simulink model "Simulaciones_de_Control"  (R2026b)
settings: Solver=ode15s  StopTime=3  MaxStep=1e-3
values from neighbouring files (symbols this model uses):
  alpha_Cu = 3.9e-3    (= 0.0039)    [coeficientes.m]
  b_eq = b_m + b_l/(r^2)    (= 2.19444444444e-05)    [coeficientes.m]
  C_ts = 0.818    [coeficientes.m]
  g = 9.80665    [coeficientes.m]
  init_I0 = 0    [coeficientes.m]
  init_Id = 0    [coeficientes.m]
  init_Iq = 0    [coeficientes.m]
  init_theta = 0    [coeficientes.m]
  init_Ts = 20    [coeficientes.m]
  init_w = 0    [coeficientes.m]
  J_eq = J_m + J_l/(r^2)    (= 4.58263888889e-05)    [coeficientes.m]
  K_et = 2*p_obs    (= 6400)    [coeficientes.m]
  K_ew = p_obs^2    (= 10240000)    [coeficientes.m]
  k_l = k_l_min + m_l*l_l    (= 1)    [coeficientes.m]
  Kd_mov = wn_mov * (2*zeta_mov + 1) * J_eq    (= 0.0916527777778)    [coeficientes.m]
  Ki_mov = wn_mov^3 * J_eq    (= 23463.1111111)    [coeficientes.m]
  Kp_mov = wn_mov^2 * (2*zeta_mov + 1) * J_eq    (= 73.3222222222)    [coeficientes.m]
  L_d = 6.6e-3    (= 0.0066)    [coeficientes.m]
  L_ls = 0.8e-3    (= 0.0008)    [coeficientes.m]
  L_q = 5.8e-3    (= 0.0058)    [coeficientes.m]
  lambda = 0.016    [coeficientes.m]
  Pp = 3    [coeficientes.m]
  r = 120.0    (= 120)    [coeficientes.m]
  R_sREF = 1.02    [coeficientes.m]
  R_tsamb = 146.7    [coeficientes.m]
  T_amb = 20    [coeficientes.m]
  T_sREF = 20    [coeficientes.m]
libraries: eeTransforms x12
(part 2 of 2)

== system Simulaciones_de_Control/Subsystem Reference1/Transformada Inversa de Park ==
  θm : Inport
  Vd : Inport  Port=2
  Vq : Inport  Port=3
  V0 : Inport  Port=4
  Bus Creator : BusCreator  Inputs=3
  Bus Creator1 : BusCreator  Inputs=3
  Demux : Demux  Outputs=3
  Gain3 : Gain  Gain=Pp
  Inverse Park Transform : eeTransforms/Inverse Park Transform  AxisAlignment=Q-axis  PowerInvariant=off
      settings: LibrarySourceBlock=|
      | ee_sl_lib/Mathematical
      | Transforms/Inverse
      | Park Transform
  Vdq0 : Outport
  Vabc : Outport  Port=2
  wires:
  Gain3/1 -> Inverse Park Transform/2
  Inverse Park Transform/1 -> Demux/1  "v_abc"
  Demux/1 -> Bus Creator/1  "Va"
  Demux/3 -> Bus Creator/3  "Vc"
  Demux/2 -> Bus Creator/2  "Vb"
  Bus Creator/1 -> Vabc/1
  θm/1 -> Gain3/1
  Vd/1 -> Bus Creator1/1
  Vq/1 -> Bus Creator1/2
  V0/1 -> Bus Creator1/3
  Bus Creator1/1 -> Vdq0/1, Inverse Park Transform/1

== system Simulaciones_de_Control/Subsystem Reference1/Transformada_Directa_de_Park_I ==
  Iabc : Inport  OutDataTypeStr=Bus: Iabc
  θm : Inport  Port=2
  Bus Creator : BusCreator  Inputs=3
  Demux : Demux  Outputs=3
  Gain3 : Gain  Gain=Pp
  Park Transform : eeTransforms/Park Transform  AxisAlignment=Q-axis  PowerInvariant=off
      settings: LibrarySourceBlock=|
      | ee_sl_lib/Mathematical
      | Transforms/Park Transform
  Idq0 : Outport  OutDataTypeStr=Bus: Idq0
  wires:
  Gain3/1 -> Park Transform/2
  Park Transform/1 -> Demux/1  "Idq0"
  Demux/1 -> Bus Creator/1  "Id"
  Demux/3 -> Bus Creator/3  "I0"
  Demux/2 -> Bus Creator/2  "Iq"
  Bus Creator/1 -> Idq0/1
  Iabc/1 -> Park Transform/1
  θm/1 -> Gain3/1

== system Simulaciones_de_Control/Subsystem Reference2/Estimador de Estado Reducido ==
  T*m : Inport
  θm : Inport  Port=2
  Gain : Gain  Gain=1/J_eq
  Gain1 : Gain  Gain=K_ew
  Gain2 : Gain  Gain=K_et
  Integrator : Integrator
  Integrator1 : Integrator
  Sum : Sum  Inputs=|++
  Sum1 : Sum  Inputs=|++
  Sum2 : Sum  Inputs=+-
  ~ωm : Outport
  ~θm : Outport  Port=2
  wires:
  T*m/1 -> Gain/1
  Gain/1 -> Sum/1
  Sum/1 -> Integrator/1  "~dωm"
  Sum1/1 -> Integrator1/1  "~ωm+e*K_et"
  Integrator/1 -> ~ωm/1, Sum1/1  "~ωm"
  Gain1/1 -> Sum/2
  Gain2/1 -> Sum1/2
  Sum2/1 -> Gain1/1, Gain2/1  "eθ"
  θm/1 -> Sum2/1  "θm"
  Integrator1/1 -> ~θm/1, Sum2/2  "~θm"

== system Simulaciones_de_Control/Subsystem Reference2/Modulador de Torque Equivalente ==
  T°s : Inport
  ωm : Inport  Port=2
  Iabc : Inport  Port=3
  θm : Inport  Port=4
  T*m : Inport  Port=5
  dinamicRs? : Inport  Port=6
  T°ref : Inport  Port=7
  Constant1 : Constant  Value=g
  Constant2 : Constant  Value=T_sREF
  Constant3 : Constant
  Gain : Gain  Gain=alpha_Cu
  Gain1 : Gain  Gain=R_sREF
  Ground : Ground
  Lazo de Control de Corrientes Virtuales : Subsystem  ReferencedSubsystem=Lazo_Corrientes
      settings: PortSchema="{\"entries\":[{\"content\":{\"sides\":[{\"content\":{\"connectorIds\":[\"In2\",\"In3\",\"In1\",\"In4\",\"In5\"]},\"type\":\"ConnectorPlacement.EquallySpacedRectSide\",\"uuid\":\"7378df2b-1b9c-42cd-9ef6-9bfa4de31228\"},{\"content\":{\"connectorIds\":[\"Out2\",\"Out1\",\"Out3\"],\"side\":\"RIGHT\"},\"type\":\"ConnectorPlacement.EquallySpacedRectSide\",\"uuid\":\"75ac4e09-b611-4ee2-aa1e-16791f3f98b8\"},{\"content\":{\"side\":\"TOP\"},\"type\":\"ConnectorPlacement.EquallySpacedRectSide\",\"uuid\":\"c32b7829-5b6a-417b-8aae-eaa4caf59bef\"}]},\"type\":\"ConnectorPlacement.EquallySpacedConnector\",\"uuid\":\"1d84f5ff-db01-492a-bfe1-22065b3eebb0\"}],\"packageUris\":[\"http://schema.mathworks.com/mf0/Connector/R2020b\"],\"version\":\"1.0\"}"
  Modulador de Tensiones Virtuales : Subsystem  ReferencedSubsystem=Modulador_Tensiones
      settings: PortSchema="{\"entries\":[{\"content\":{\"sides\":[{\"content\":{\"connectorIds\":[\"In2\",\"In1\",\"In3\",\"In6\",\"In7\",\"In5\",\"In4\"]},\"type\":\"ConnectorPlacement.EquallySpacedRectSide\",\"uuid\":\"561a625a-719f-47d4-85d3-a88e423068dd\"},{\"content\":{\"connectorIds\":[\"Out2\",\"Out1\"],\"side\":\"RIGHT\"},\"type\":\"ConnectorPlacement.EquallySpacedRectSide\",\"uuid\":\"c1cdd74a-6c1d-470e-a6ac-8d72e83b5cc5\"},{\"content\":{\"side\":\"TOP\"},\"type\":\"ConnectorPlacement.EquallySpacedRectSide\",\"uuid\":\"c5935c6f-534c-46b9-aa64-6d6dabbbb210\"}]},\"type\":\"ConnectorPlacement.EquallySpacedConnector\",\"uuid\":\"b0debde9-6e18-4e06-b0c4-28c9c51e472d\"}],\"packageUris\":[\"http://schema.mathworks.com/mf0/Connector/R2020b\"],\"version\":\"1.0\"}"
  Modulador y Compensación de Torque : Subsystem  ReferencedSubsystem=Lazo_Torque
      settings: PortSchema="{\"entries\":[{\"content\":{\"sides\":[{\"content\":{\"connectorIds\":[\"In5\",\"In1\",\"In2\",\"In3\",\"In4\"]},\"type\":\"ConnectorPlacement.EquallySpacedRectSide\",\"uuid\":\"ea9ad4ab-f607-4d37-9442-85f6cfda2486\"},{\"content\":{\"connectorIds\":[\"Out1\"],\"side\":\"RIGHT\"},\"type\":\"ConnectorPlacement.EquallySpacedRectSide\",\"uuid\":\"696b5fe5-1f6c-4fc9-932e-86b56d49996f\"},{\"content\":{\"side\":\"TOP\"},\"type\":\"ConnectorPlacement.EquallySpacedRectSide\",\"uuid\":\"45e3ac4c-5a2f-4a79-9454-e497b07295c7\"}]},\"type\":\"ConnectorPlacement.EquallySpacedConnector\",\"uuid\":\"ad401c21-3c60-4ab4-96eb-f449fc93609a\"}],\"packageUris\":[\"http://schema.mathworks.com/mf0/Connector/R2020b\"],\"version\":\"1.0\"}"
  Subsystem : Subsystem
  Sum : Sum  Inputs=|+-
  Sum1 : Sum  Inputs=|++
  Switch : Switch  Criteria=u2 > Threshold  SaturateOnIntegerOverflow=off  InputSameDT=off
  Vabc : Outport
  Vdq0 : Outport  Port=2
  wires:
  Sum1/1 -> Gain1/1
  Constant3/1 -> Sum1/2
  Gain/1 -> Sum1/1
  Sum/1 -> Gain/1
  Constant2/1 -> Sum/2
  T°ref/1 -> Sum/1
  Constant1/1 -> Modulador y Compensación de Torque/5
  Modulador de Tensiones Virtuales/2 -> Vdq0/1
  Gain1/1 -> Switch/3
  Switch/1 -> Modulador de Tensiones Virtuales/4  "Rs"
  dinamicRs?/1 -> Switch/2  "True_False"
  Subsystem/1(R_s) -> Switch/1  "Rs"
  T°s/1 -> Subsystem/1(T°s)
  Iabc/1 -> Modulador y Compensación de Torque/2, Lazo de Control de Corrientes Virtuales/4, Modulador de Tensiones Virtuales/6  "Iabc"
  Ground/1 -> Lazo de Control de Corrientes Virtuales/3, Lazo de Control de Corrientes Virtuales/2
  Modulador de Tensiones Virtuales/1 -> Vabc/1
  ωm/1 -> Modulador y Compensación de Torque/4, Modulador de Tensiones Virtuales/5  "ωm"
  θm/1 -> Modulador y Compensación de Torque/3, Lazo de Control de Corrientes Virtuales/5, Modulador de Tensiones Virtuales/7  "θm"
  T*m/1 -> Modulador y Compensación de Torque/1
  Modulador y Compensación de Torque/1 -> Lazo de Control de Corrientes Virtuales/1
  Lazo de Control de Corrientes Virtuales/3 -> Modulador de Tensiones Virtuales/3
  Lazo de Control de Corrientes Virtuales/2 -> Modulador de Tensiones Virtuales/2
  Lazo de Control de Corrientes Virtuales/1 -> Modulador de Tensiones Virtuales/1

== system Simulaciones_de_Control/Subsystem Reference2/PID Movimiento ==
  ωm : Inport  Unit=rad/s
  θm : Inport  Port=2
  θm* : Inport  Port=3  Unit=rad/s
  ωm* : Inport  Port=4  Unit=rad/s
  Gain : Gain  Gain=Kd_mov
  Gain1 : Gain  Gain=Kp_mov
  Gain2 : Gain  Gain=Ki_mov
  Integrator1 : Integrator
  Sum : Sum  Inputs=|+-
  Sum1 : Sum  Inputs=+++
  Sum2 : Sum  Inputs=|+-
  T*m : Outport
  wires:
  Gain1/1 -> Sum1/2
  Sum1/1 -> T*m/1
  Gain2/1 -> Sum1/1
  Gain/1 -> Sum1/3
  θm*/1 -> Sum2/1
  Sum/1 -> Gain/1  "eω"
  θm/1 -> Sum2/2
  ωm*/1 -> Sum/1
  ωm/1 -> Sum/2
  Integrator1/1 -> Gain2/1  "e∫θ"
  Sum2/1 -> Gain1/1, Integrator1/1  "eθ"

== system Simulaciones_de_Control/Subsystem Reference2/Planta (Modelo Global No Lineal) ==
  note: Sistema Global No Lineal
  Vabc : Inport  OutDataTypeStr=Bus: Vabc
  T_ld : Inport  Port=2
  g : Inport  Port=3
  T°amb : Inport  Port=4
  Id(0) : Inport  Port=5
  Bus Selector : BusSelector  OutputSignals=Vd,Vq,V0
  Gain : Gain  Gain=Pp
  Subsistema Electromagnetico : Subsystem
  Subsistema Mecanico Equivalente : Subsystem
  Subsistema Termico : Subsystem
  Transformada Directa de Park : Subsystem
  Transformada Inversa de Park : Subsystem  ReferencedSubsystem=Transformada_Inversa_de_Park_I
  θm : Outport
  Iabc : Outport  Port=2  OutDataTypeStr=Bus: Iabc
  T°s : Outport  Port=3
  ωm : Outport  Port=4
  Tm : Outport  Port=5
  wires:
  Id(0)/1 -> Subsistema Electromagnetico/6(Id(0))
  Transformada Inversa de Park/1 -> Iabc/1  "Iabc"
  Bus Selector/3 -> Subsistema Electromagnetico/5(V0)  "<V0>"
  Bus Selector/2 -> Subsistema Electromagnetico/4(Vq)  "<Vq>"
  Bus Selector/1 -> Subsistema Electromagnetico/3(Vd)  "<Vd>"
  Transformada Directa de Park/1(Vdq0) -> Bus Selector/1
  g/1 -> Subsistema Mecanico Equivalente/3(g)
  T°amb/1 -> Subsistema Termico/2(T°amb)
  Vabc/1 -> Transformada Directa de Park/1(Vabc)
  T_ld/1 -> Subsistema Mecanico Equivalente/2(T_ld)
  Gain/1 -> Subsistema Electromagnetico/2(ωr)
  Subsistema Termico/1(R_s) -> Subsistema Electromagnetico/1(R_s)
  Subsistema Electromagnetico/2(T_m) -> Tm/1, Subsistema Mecanico Equivalente/1(T_m)  "Tm"
  Subsistema Mecanico Equivalente/2(θm) -> θm/1, Transformada Inversa de Park/2, Transformada Directa de Park/2(θm)  "θm"
  Subsistema Mecanico Equivalente/1(ωm) -> ωm/1, Gain/1  "ωm"
  Subsistema Electromagnetico/1(Idq0) -> Transformada Inversa de Park/1, Subsistema Termico/1(Idq0)  "Idq0"
  Subsistema Termico/2(T°s) -> T°s/1  "T°s"

== system Simulaciones_de_Control/Subsystem Reference2/Sensores Ideales ==
  note: RTD
  note: Amperimetros
  note: Encoder
  θm : Inport
  Iabc : Inport  Port=2
  T°s : Inport  Port=3
  Bus Creator : BusCreator  Inputs=3
  Bus Selector : BusSelector  OutputSignals=Ia,Ib,Ic
  Gain{,1..4} (5 alike) : Gain
  θm' : Outport
  Iabc' : Outport  Port=2
  T°s' : Outport  Port=3
  wires:
  Gain3/1 -> Bus Creator/3  "Ic"
  Gain1/1 -> Bus Creator/1  "Ia"
  Gain2/1 -> Bus Creator/2  "Ib"
  Bus Selector/3 -> Gain3/1  "<Ic>"
  Bus Selector/2 -> Gain2/1  "<Ib>"
  Bus Selector/1 -> Gain1/1  "<Ia>"
  Iabc/1 -> Bus Selector/1
  Bus Creator/1 -> Iabc'/1
  Gain4/1 -> T°s'/1
  T°s/1 -> Gain4/1
  Gain/1 -> θm'/1
  θm/1 -> Gain/1

== system Simulaciones_de_Control/Subsystem Reference2/Transformada_Directa_de_Park_I ==
  Iabc : Inport  OutDataTypeStr=Bus: Iabc
  θm : Inport  Port=2
  Ancho_abc : SignalSpecification  Dimensions=3
  Bus Creator : BusCreator  Inputs=3
  Bus to Vector : BusToVector
  Demux : Demux  Outputs=3
  Gain3 : Gain  Gain=Pp
  Park Transform : eeTransforms/Park Transform  AxisAlignment=Q-axis  PowerInvariant=off
      settings: LibrarySourceBlock=|
      | ee_sl_lib/Mathematical
      | Transforms/Park Transform
  Idq0 : Outport  OutDataTypeStr=Bus: Idq0
  wires:
  Ancho_abc/1 -> Park Transform/1
  Bus to Vector/1 -> Ancho_abc/1
  θm/1 -> Gain3/1
  Iabc/1 -> Bus to Vector/1
  Bus Creator/1 -> Idq0/1
  Demux/2 -> Bus Creator/2  "Iq"
  Demux/3 -> Bus Creator/3  "I0"
  Demux/1 -> Bus Creator/1  "Id"
  Park Transform/1 -> Demux/1  "Idq0"
  Gain3/1 -> Park Transform/2

== system Simulaciones_de_Control/Simulacion Modulador de Tension/Modulador de Tensiones Virtuales/Transformada Directa de Park ==
  Iabc : Inport
  θm : Inport  Port=2
  Bus Creator : BusCreator  Inputs=3
  Demux : Demux  Outputs=3
  Gain3 : Gain  Gain=Pp
  Park Transform : eeTransforms/Park Transform  AxisAlignment=Q-axis  PowerInvariant=off
      settings: LibrarySourceBlock=|
      | ee_sl_lib/Mathematical
      | Transforms/Park Transform
  Idq0 : Outport
  wires:
  Gain3/1 -> Park Transform/2
  Park Transform/1 -> Demux/1  "Idq0"
  Demux/1 -> Bus Creator/1  "Id"
  Demux/3 -> Bus Creator/3  "I0"
  Demux/2 -> Bus Creator/2  "Iq"
  Bus Creator/1 -> Idq0/1
  Iabc/1 -> Park Transform/1
  θm/1 -> Gain3/1

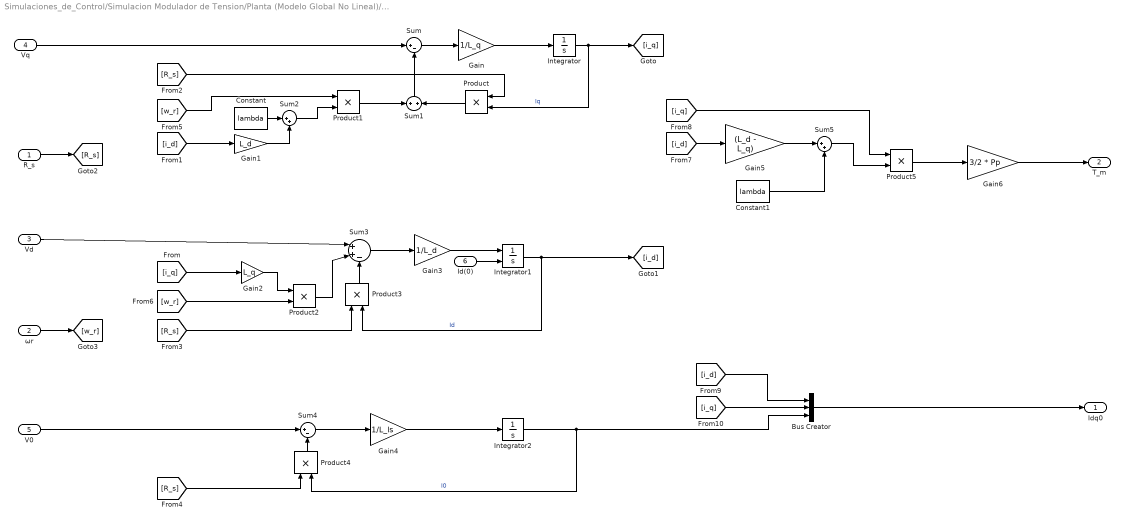
== system Simulaciones_de_Control/Simulacion Modulador de Tension/Planta (Modelo Global No Lineal)/Subsistema Electromagnetico ==
  R_s : Inport
  ωr : Inport  Port=2
  Vd : Inport  Port=3
  Vq : Inport  Port=4
  V0 : Inport  Port=5
  Id(0) : Inport  Port=6
  Bus Creator : BusCreator  Inputs=3
  Constant : Constant  Value=lambda
  Constant1 : Constant  Value=lambda
  Gain : Gain  Gain=1/L_q
  Gain1 : Gain  Gain=L_d
  Gain2 : Gain  Gain=L_q
  Gain3 : Gain  Gain=1/L_d
  Gain4 : Gain  Gain=1/L_ls
  Gain5 : Gain  Gain=(L_d - L_q)
  Gain6 : Gain  Gain=3/2 * Pp
  Integrator : Integrator  InitialCondition=init_Iq
  Integrator1 : Integrator  InitialConditionSource=external  InitialCondition=init_Id
  Integrator2 : Integrator  InitialCondition=init_I0
  Product{,1..5} (6 alike) : Product
  Sum : Sum  Inputs=|+-
  Sum1 : Sum
  Sum2 : Sum  Inputs=|++
  Sum3 : Sum  Inputs=|++-
  Sum4 : Sum  Inputs=|+-
  Sum5 : Sum  Inputs=|++
  Idq0 : Outport
  T_m : Outport  Port=2
  wires:
  [i_q] -> Bus Creator/2
  [i_d] -> Bus Creator/1
  Id(0)/1 -> Integrator1/2
  Bus Creator/1 -> Idq0/1
  [i_q] -> Product5/1
  [i_d] -> Gain5/1
  [w_r] -> Product1/1
  ωr/1 -> [w_r]
  [R_s] -> Product4/1
  [R_s] -> Product3/1
  R_s/1 -> [R_s]
  [i_d] -> Gain1/1
  Gain6/1 -> T_m/1
  Product5/1 -> Gain6/1
  Constant1/1 -> Sum5/2
  Integrator1/1 -> Product3/2, [i_d]  "Id"
  Sum5/1 -> Product5/2
  Gain5/1 -> Sum5/1
  V0/1 -> Sum4/1
  Sum4/1 -> Gain4/1
  Gain4/1 -> Integrator2/1
  Integrator2/1 -> Product4/2, Bus Creator/3  "I0"
  Product4/1 -> Sum4/2
  Vd/1 -> Sum3/1
  Sum3/1 -> Gain3/1
  Gain3/1 -> Integrator1/1
  Product3/1 -> Sum3/3
  Gain/1 -> Integrator/1
  Vq/1 -> Sum/1
  Sum/1 -> Gain/1
  Constant/1 -> Sum2/1
  Sum2/1 -> Product1/2
  Gain1/1 -> Sum2/2
  Product1/1 -> Sum1/1
  Sum1/1 -> Sum/2
  Product/1 -> Sum1/2
  [R_s] -> Product/1
  Integrator/1 -> [i_q], Product/2  "Iq"
  [i_q] -> Gain2/1
  Product2/1 -> Sum3/2
  Gain2/1 -> Product2/1
  [w_r] -> Product2/2

== system Simulaciones_de_Control/Simulacion Modulador de Tension/Planta (Modelo Global No Lineal)/Subsistema Mecanico Equivalente ==
  note: $\theta_m$
  note: $\omega_m$
  note: $\dot{\omega}_m$
  note: $T_{ld}$
  note: $T_m$
  T_m : Inport
  T_ld : Inport  Port=2
  g : Inport  Port=3
  Gain : Gain  Gain=1/r
  Gain1 : Gain  Gain=b_eq
  Gain2 : Gain  Gain=k_l/r
  Gain3 : Gain  Gain=1/J_eq
  Gain4 : Gain  Gain=1/r
  Integrator : Integrator  InitialCondition=init_w
  Integrator1 : Integrator  InitialCondition=init_theta
  Product : Product
  Sin : Trigonometry
  Sum : Sum  Inputs=|+-
  Sum1 : Sum  Inputs=+++
  ωm : Outport
  θm : Outport  Port=2
  wires:
  Integrator1/1 -> θm/1, Gain4/1
  Integrator/1 -> Gain1/1, Integrator1/1, ωm/1
  g/1 -> Product/1
  Product/1 -> Sum1/2
  T_ld/1 -> Gain/1
  Gain4/1 -> Sin/1
  Gain3/1 -> Integrator/1
  Gain1/1 -> Sum1/3
  Sin/1 -> Gain2/1
  Gain/1 -> Sum1/1
  Gain2/1 -> Product/2
  Sum1/1 -> Sum/2
  T_m/1 -> Sum/1
  Sum/1 -> Gain3/1

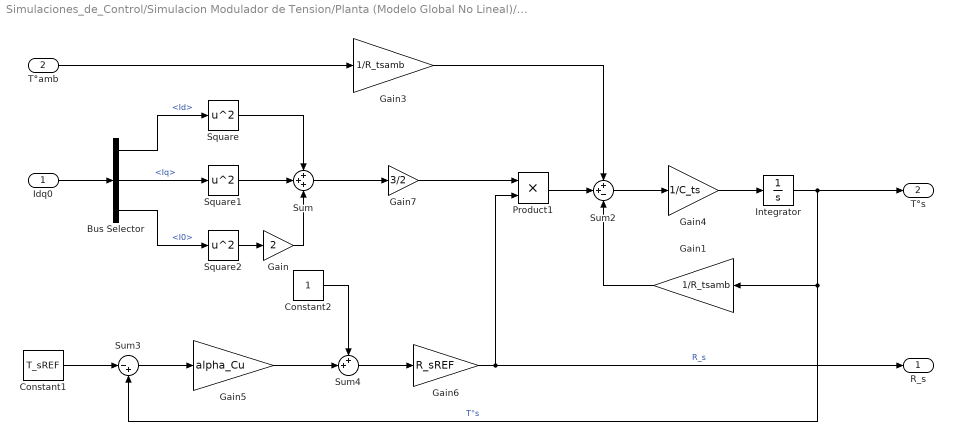
== system Simulaciones_de_Control/Simulacion Modulador de Tension/Planta (Modelo Global No Lineal)/Subsistema Termico ==
  Idq0 : Inport
  T°amb : Inport  Port=2
  Bus Selector : BusSelector  OutputSignals=Id,Iq,I0
  Constant1 : Constant  Value=T_sREF
  Constant2 : Constant
  Gain : Gain  Gain=2
  Gain1 : Gain  Gain=1/R_tsamb
  Gain3 : Gain  Gain=1/R_tsamb
  Gain4 : Gain  Gain=1/C_ts
  Gain5 : Gain  Gain=alpha_Cu
  Gain6 : Gain  Gain=R_sREF
  Gain7 : Gain  Gain=3/2
  Integrator : Integrator  InitialCondition=init_Ts
  Product1 : Product
  Square : Math  Operator=square
  Square1 : Math  Operator=square
  Square2 : Math  Operator=square
  Sum : Sum  Inputs=+++
  Sum2 : Sum  Inputs=++-
  Sum3 : Sum  Inputs=|-+
  Sum4 : Sum  Inputs=++|
  R_s : Outport
  T°s : Outport  Port=2
  wires:
  Bus Selector/3 -> Square2/1  "<I0>"
  Bus Selector/1 -> Square/1  "<Id>"
  Constant2/1 -> Sum4/1
  Idq0/1 -> Bus Selector/1
  Gain3/1 -> Sum2/1
  Gain1/1 -> Sum2/3
  Gain4/1 -> Integrator/1
  Product1/1 -> Sum2/2
  Square/1 -> Sum/1
  Sum2/1 -> Gain4/1
  Square2/1 -> Gain/1
  Sum/1 -> Gain7/1
  T°amb/1 -> Gain3/1
  Sum3/1 -> Gain5/1
  Gain5/1 -> Sum4/2
  Gain/1 -> Sum/3
  Constant1/1 -> Sum3/1
  Sum4/1 -> Gain6/1
  Gain7/1 -> Product1/1
  Gain6/1 -> Product1/2, R_s/1  "R_s"
  Integrator/1 -> T°s/1, Gain1/1, Sum3/2  "T°s"
  Square1/1 -> Sum/2
  Bus Selector/2 -> Square1/1  "<Iq>"

== system Simulaciones_de_Control/Subsystem Reference/Modulador de Torque Equivalente/Subsystem ==
  T°s : Inport
  Constant1 : Constant  Value=T_sREF
  Constant2 : Constant
  Gain5 : Gain  Gain=alpha_Cu
  Gain6 : Gain  Gain=R_sREF
  Sum3 : Sum  Inputs=+-|
  Sum4 : Sum  Inputs=|++
  R_s : Outport
  wires:
  T°s/1 -> Sum3/1
  Gain5/1 -> Sum4/1
  Gain6/1 -> R_s/1  "R_s"
  Constant1/1 -> Sum3/2
  Constant2/1 -> Sum4/2
  Sum4/1 -> Gain6/1
  Sum3/1 -> Gain5/1

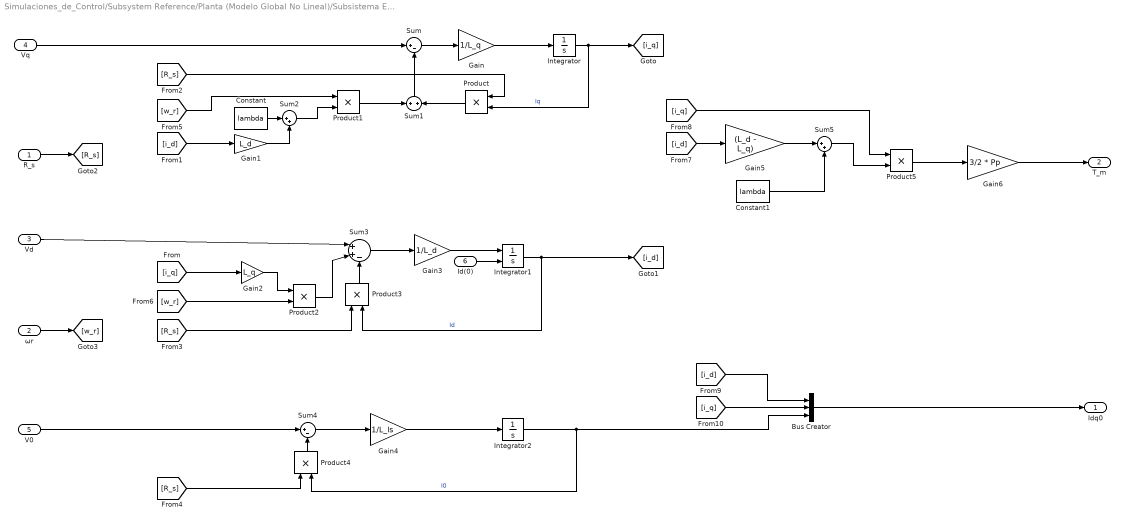
== system Simulaciones_de_Control/Subsystem Reference/Planta (Modelo Global No Lineal)/Subsistema Electromagnetico ==
  R_s : Inport
  ωr : Inport  Port=2
  Vd : Inport  Port=3
  Vq : Inport  Port=4
  V0 : Inport  Port=5
  Id(0) : Inport  Port=6
  Bus Creator : BusCreator  Inputs=3
  Constant : Constant  Value=lambda
  Constant1 : Constant  Value=lambda
  Gain : Gain  Gain=1/L_q
  Gain1 : Gain  Gain=L_d
  Gain2 : Gain  Gain=L_q
  Gain3 : Gain  Gain=1/L_d
  Gain4 : Gain  Gain=1/L_ls
  Gain5 : Gain  Gain=(L_d - L_q)
  Gain6 : Gain  Gain=3/2 * Pp
  Integrator : Integrator  InitialCondition=init_Iq
  Integrator1 : Integrator  InitialConditionSource=external  InitialCondition=init_Id
  Integrator2 : Integrator  InitialCondition=init_I0
  Product{,1..5} (6 alike) : Product
  Sum : Sum  Inputs=|+-
  Sum1 : Sum
  Sum2 : Sum  Inputs=|++
  Sum3 : Sum  Inputs=|++-
  Sum4 : Sum  Inputs=|+-
  Sum5 : Sum  Inputs=|++
  Idq0 : Outport
  T_m : Outport  Port=2
  wires:
  [w_r] -> Product2/2
  Gain2/1 -> Product2/1
  Product2/1 -> Sum3/2
  [i_q] -> Gain2/1
  Integrator/1 -> Product/2, [i_q]  "Iq"
  [R_s] -> Product/1
  Product/1 -> Sum1/2
  Sum1/1 -> Sum/2
  Product1/1 -> Sum1/1
  Gain1/1 -> Sum2/2
  Sum2/1 -> Product1/2
  Constant/1 -> Sum2/1
  Sum/1 -> Gain/1
  Vq/1 -> Sum/1
  Gain/1 -> Integrator/1
  Product3/1 -> Sum3/3
  Gain3/1 -> Integrator1/1
  Sum3/1 -> Gain3/1
  Vd/1 -> Sum3/1
  Product4/1 -> Sum4/2
  Integrator2/1 -> Bus Creator/3, Product4/2  "I0"
  Gain4/1 -> Integrator2/1
  Sum4/1 -> Gain4/1
  V0/1 -> Sum4/1
  Gain5/1 -> Sum5/1
  Sum5/1 -> Product5/2
  Integrator1/1 -> [i_d], Product3/2  "Id"
  Constant1/1 -> Sum5/2
  Product5/1 -> Gain6/1
  Gain6/1 -> T_m/1
  [i_d] -> Gain1/1
  R_s/1 -> [R_s]
  [R_s] -> Product3/1
  [R_s] -> Product4/1
  ωr/1 -> [w_r]
  [w_r] -> Product1/1
  [i_d] -> Gain5/1
  [i_q] -> Product5/1
  Bus Creator/1 -> Idq0/1
  Id(0)/1 -> Integrator1/2
  [i_d] -> Bus Creator/1
  [i_q] -> Bus Creator/2

== system Simulaciones_de_Control/Subsystem Reference/Planta (Modelo Global No Lineal)/Subsistema Mecanico Equivalente ==
  note: $T_m$
  note: $T_{ld}$
  note: $\dot{\omega}_m$
  note: $\omega_m$
  note: $\theta_m$
  T_m : Inport
  T_ld : Inport  Port=2
  g : Inport  Port=3
  Gain : Gain  Gain=1/r
  Gain1 : Gain  Gain=b_eq
  Gain2 : Gain  Gain=k_l/r
  Gain3 : Gain  Gain=1/J_eq
  Gain4 : Gain  Gain=1/r
  Integrator : Integrator  InitialCondition=init_w
  Integrator1 : Integrator  InitialCondition=init_theta
  Product : Product
  Sin : Trigonometry
  Sum : Sum  Inputs=|+-
  Sum1 : Sum  Inputs=+++
  ωm : Outport
  θm : Outport  Port=2
  wires:
  Sum/1 -> Gain3/1
  T_m/1 -> Sum/1
  Sum1/1 -> Sum/2
  Gain2/1 -> Product/2
  Gain/1 -> Sum1/1
  Sin/1 -> Gain2/1
  Gain1/1 -> Sum1/3
  Gain3/1 -> Integrator/1
  Gain4/1 -> Sin/1
  T_ld/1 -> Gain/1
  Product/1 -> Sum1/2
  g/1 -> Product/1
  Integrator/1 -> ωm/1, Integrator1/1, Gain1/1
  Integrator1/1 -> Gain4/1, θm/1

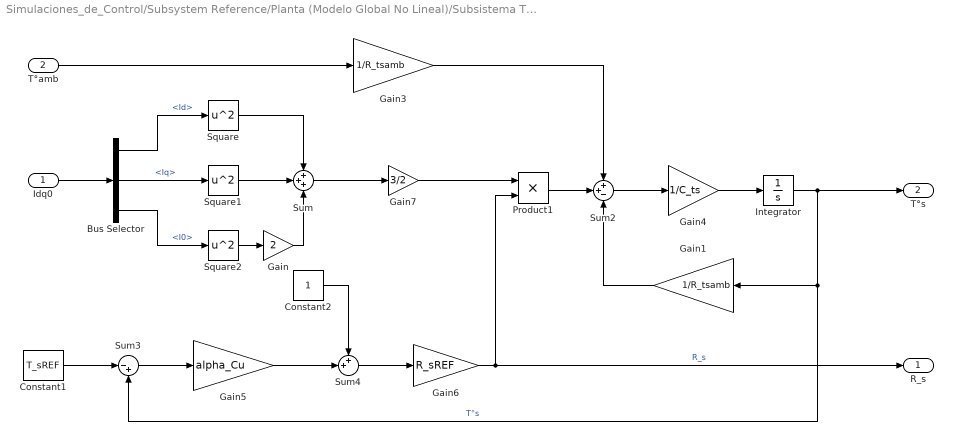
== system Simulaciones_de_Control/Subsystem Reference/Planta (Modelo Global No Lineal)/Subsistema Termico ==
  Idq0 : Inport
  T°amb : Inport  Port=2
  Bus Selector : BusSelector  OutputSignals=Id,Iq,I0
  Constant1 : Constant  Value=T_sREF
  Constant2 : Constant
  Gain : Gain  Gain=2
  Gain1 : Gain  Gain=1/R_tsamb
  Gain3 : Gain  Gain=1/R_tsamb
  Gain4 : Gain  Gain=1/C_ts
  Gain5 : Gain  Gain=alpha_Cu
  Gain6 : Gain  Gain=R_sREF
  Gain7 : Gain  Gain=3/2
  Integrator : Integrator  InitialCondition=init_Ts
  Product1 : Product
  Square : Math  Operator=square
  Square1 : Math  Operator=square
  Square2 : Math  Operator=square
  Sum : Sum  Inputs=+++
  Sum2 : Sum  Inputs=++-
  Sum3 : Sum  Inputs=|-+
  Sum4 : Sum  Inputs=++|
  R_s : Outport
  T°s : Outport  Port=2
  wires:
  Bus Selector/2 -> Square1/1  "<Iq>"
  Square1/1 -> Sum/2
  Integrator/1 -> Sum3/2, Gain1/1, T°s/1  "T°s"
  Gain6/1 -> R_s/1, Product1/2  "R_s"
  Gain7/1 -> Product1/1
  Sum4/1 -> Gain6/1
  Constant1/1 -> Sum3/1
  Gain/1 -> Sum/3
  Gain5/1 -> Sum4/2
  Sum3/1 -> Gain5/1
  T°amb/1 -> Gain3/1
  Sum/1 -> Gain7/1
  Square2/1 -> Gain/1
  Sum2/1 -> Gain4/1
  Square/1 -> Sum/1
  Product1/1 -> Sum2/2
  Gain4/1 -> Integrator/1
  Gain1/1 -> Sum2/3
  Gain3/1 -> Sum2/1
  Idq0/1 -> Bus Selector/1
  Constant2/1 -> Sum4/1
  Bus Selector/1 -> Square/1  "<Id>"
  Bus Selector/3 -> Square2/1  "<I0>"

== system Simulaciones_de_Control/Subsystem Reference/Planta (Modelo Global No Lineal)/Transformada Directa de Park ==
  Vabc : Inport  OutDataTypeStr=Bus: Vabc
  θm : Inport  Port=2
  Bus Creator : BusCreator  Inputs=3
  Demux : Demux  Outputs=3
  Gain3 : Gain  Gain=Pp
  MATLAB Function2 : MATLAB Function  Commented=on  TreatAsAtomicUnit=on
  Park Transform : eeTransforms/Park Transform  AxisAlignment=Q-axis  PowerInvariant=off
      settings: LibrarySourceBlock=|
      | ee_sl_lib/Mathematical
      | Transforms/Park Transform
  Vdq0 : Outport  OutDataTypeStr=Bus: Vdq0
  wires:
  Vabc/1 -> Park Transform/1
  Park Transform/1 -> Demux/1  "v_dq0"
  θm/1 -> Gain3/1
  Bus Creator/1 -> Vdq0/1
  Demux/2 -> Bus Creator/2  "Vq"
  Demux/3 -> Bus Creator/3  "V0"
  Demux/1 -> Bus Creator/1  "Vd"
  Gain3/1 -> Park Transform/2

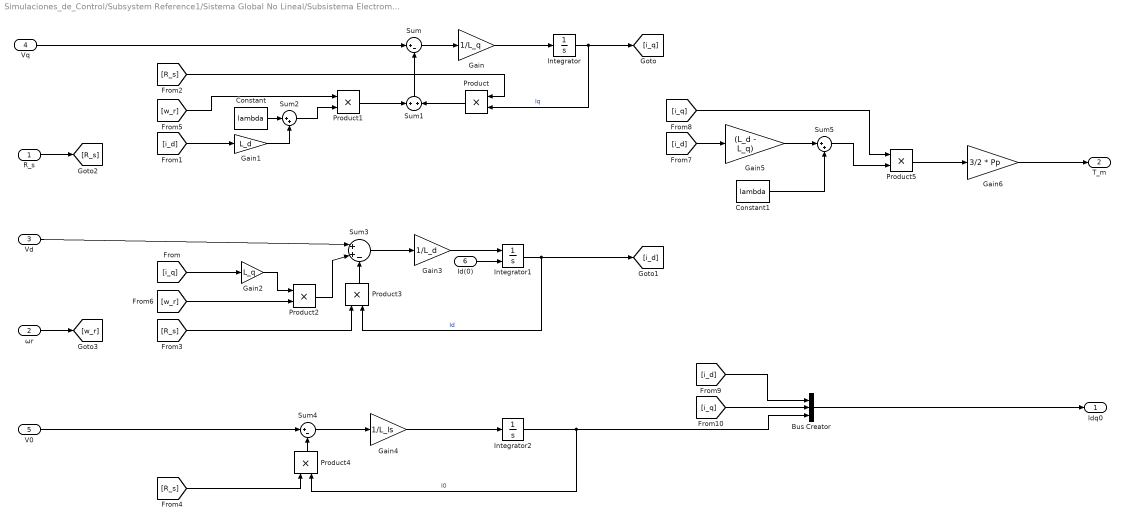
== system Simulaciones_de_Control/Subsystem Reference1/Sistema Global No Lineal/Subsistema Electromagnetico ==
  R_s : Inport
  ωr : Inport  Port=2
  Vd : Inport  Port=3
  Vq : Inport  Port=4
  V0 : Inport  Port=5
  Id(0) : Inport  Port=6
  Bus Creator : BusCreator  Inputs=3
  Constant : Constant  Value=lambda
  Constant1 : Constant  Value=lambda
  Gain : Gain  Gain=1/L_q
  Gain1 : Gain  Gain=L_d
  Gain2 : Gain  Gain=L_q
  Gain3 : Gain  Gain=1/L_d
  Gain4 : Gain  Gain=1/L_ls
  Gain5 : Gain  Gain=(L_d - L_q)
  Gain6 : Gain  Gain=3/2 * Pp
  Integrator : Integrator  InitialCondition=init_Iq
  Integrator1 : Integrator  InitialConditionSource=external  InitialCondition=init_Id
  Integrator2 : Integrator  InitialCondition=init_I0
  Product{,1..5} (6 alike) : Product
  Sum : Sum  Inputs=|+-
  Sum1 : Sum
  Sum2 : Sum  Inputs=|++
  Sum3 : Sum  Inputs=|++-
  Sum4 : Sum  Inputs=|+-
  Sum5 : Sum  Inputs=|++
  Idq0 : Outport
  T_m : Outport  Port=2
  wires:
  [w_r] -> Product2/2
  Gain2/1 -> Product2/1
  Product2/1 -> Sum3/2
  [i_q] -> Gain2/1
  Integrator/1 -> Product/2, [i_q]  "Iq"
  [R_s] -> Product/1
  Product/1 -> Sum1/2
  Sum1/1 -> Sum/2
  Product1/1 -> Sum1/1
  Gain1/1 -> Sum2/2
  Sum2/1 -> Product1/2
  Constant/1 -> Sum2/1
  Sum/1 -> Gain/1
  Vq/1 -> Sum/1
  Gain/1 -> Integrator/1
  Product3/1 -> Sum3/3
  Gain3/1 -> Integrator1/1
  Sum3/1 -> Gain3/1
  Vd/1 -> Sum3/1
  Product4/1 -> Sum4/2
  Integrator2/1 -> Bus Creator/3, Product4/2  "I0"
  Gain4/1 -> Integrator2/1
  Sum4/1 -> Gain4/1
  V0/1 -> Sum4/1
  Gain5/1 -> Sum5/1
  Sum5/1 -> Product5/2
  Integrator1/1 -> [i_d], Product3/2  "Id"
  Constant1/1 -> Sum5/2
  Product5/1 -> Gain6/1
  Gain6/1 -> T_m/1
  [i_d] -> Gain1/1
  R_s/1 -> [R_s]
  [R_s] -> Product3/1
  [R_s] -> Product4/1
  ωr/1 -> [w_r]
  [w_r] -> Product1/1
  [i_d] -> Gain5/1
  [i_q] -> Product5/1
  Bus Creator/1 -> Idq0/1
  Id(0)/1 -> Integrator1/2
  [i_d] -> Bus Creator/1
  [i_q] -> Bus Creator/2

== system Simulaciones_de_Control/Subsystem Reference1/Sistema Global No Lineal/Subsistema Mecanico Equivalente ==
  note: $T_m$
  note: $T_{ld}$
  note: $\dot{\omega}_m$
  note: $\omega_m$
  note: $\theta_m$
  T_m : Inport
  T_ld : Inport  Port=2
  g : Inport  Port=3
  Gain : Gain  Gain=1/r
  Gain1 : Gain  Gain=b_eq
  Gain2 : Gain  Gain=k_l/r
  Gain3 : Gain  Gain=1/J_eq
  Gain4 : Gain  Gain=1/r
  Integrator : Integrator  InitialCondition=init_w
  Integrator1 : Integrator  InitialCondition=init_theta
  Product : Product
  Sin : Trigonometry
  Sum : Sum  Inputs=|+-
  Sum1 : Sum  Inputs=+++
  ωm : Outport
  θm : Outport  Port=2
  wires:
  Sum/1 -> Gain3/1
  T_m/1 -> Sum/1
  Sum1/1 -> Sum/2
  Gain2/1 -> Product/2
  Gain/1 -> Sum1/1
  Sin/1 -> Gain2/1
  Gain1/1 -> Sum1/3
  Gain3/1 -> Integrator/1
  Gain4/1 -> Sin/1
  T_ld/1 -> Gain/1
  Product/1 -> Sum1/2
  g/1 -> Product/1
  Integrator/1 -> ωm/1, Integrator1/1, Gain1/1
  Integrator1/1 -> Gain4/1, θm/1

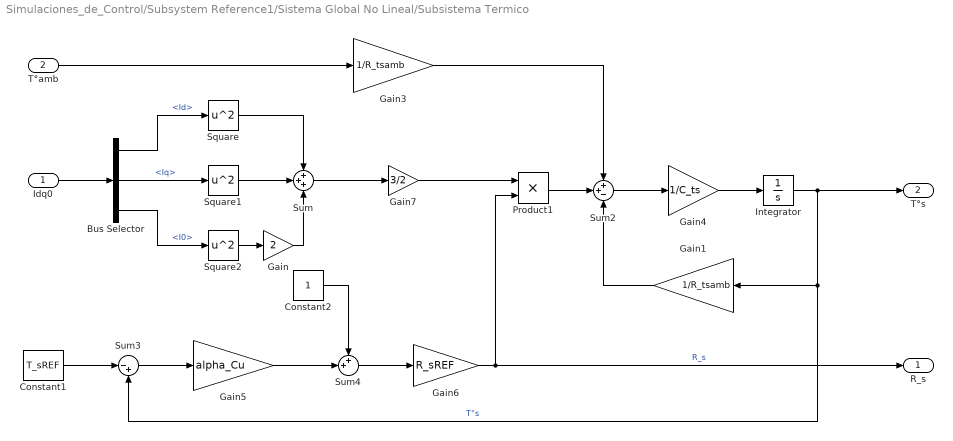
== system Simulaciones_de_Control/Subsystem Reference1/Sistema Global No Lineal/Subsistema Termico ==
  Idq0 : Inport
  T°amb : Inport  Port=2
  Bus Selector : BusSelector  OutputSignals=Id,Iq,I0
  Constant1 : Constant  Value=T_sREF
  Constant2 : Constant
  Gain : Gain  Gain=2
  Gain1 : Gain  Gain=1/R_tsamb
  Gain3 : Gain  Gain=1/R_tsamb
  Gain4 : Gain  Gain=1/C_ts
  Gain5 : Gain  Gain=alpha_Cu
  Gain6 : Gain  Gain=R_sREF
  Gain7 : Gain  Gain=3/2
  Integrator : Integrator  InitialCondition=init_Ts
  Product1 : Product
  Square : Math  Operator=square
  Square1 : Math  Operator=square
  Square2 : Math  Operator=square
  Sum : Sum  Inputs=+++
  Sum2 : Sum  Inputs=++-
  Sum3 : Sum  Inputs=|-+
  Sum4 : Sum  Inputs=++|
  R_s : Outport
  T°s : Outport  Port=2
  wires:
  Bus Selector/2 -> Square1/1  "<Iq>"
  Square1/1 -> Sum/2
  Integrator/1 -> Sum3/2, Gain1/1, T°s/1  "T°s"
  Gain6/1 -> R_s/1, Product1/2  "R_s"
  Gain7/1 -> Product1/1
  Sum4/1 -> Gain6/1
  Constant1/1 -> Sum3/1
  Gain/1 -> Sum/3
  Gain5/1 -> Sum4/2
  Sum3/1 -> Gain5/1
  T°amb/1 -> Gain3/1
  Sum/1 -> Gain7/1
  Square2/1 -> Gain/1
  Sum2/1 -> Gain4/1
  Square/1 -> Sum/1
  Product1/1 -> Sum2/2
  Gain4/1 -> Integrator/1
  Gain1/1 -> Sum2/3
  Gain3/1 -> Sum2/1
  Idq0/1 -> Bus Selector/1
  Constant2/1 -> Sum4/1
  Bus Selector/1 -> Square/1  "<Id>"
  Bus Selector/3 -> Square2/1  "<I0>"

== system Simulaciones_de_Control/Subsystem Reference1/Sistema Global No Lineal/Transformada Directa de Park ==
  Vabc : Inport  OutDataTypeStr=Bus: Vabc
  θm : Inport  Port=2
  Bus Creator : BusCreator  Inputs=3
  Demux : Demux  Outputs=3
  Gain3 : Gain  Gain=Pp
  MATLAB Function2 : MATLAB Function  Commented=on  TreatAsAtomicUnit=on
  Park Transform : eeTransforms/Park Transform  AxisAlignment=Q-axis  PowerInvariant=off
      settings: LibrarySourceBlock=|
      | ee_sl_lib/Mathematical
      | Transforms/Park Transform
  Vdq0 : Outport  OutDataTypeStr=Bus: Vdq0
  wires:
  Gain3/1 -> Park Transform/2
  Demux/1 -> Bus Creator/1  "Vd"
  Demux/3 -> Bus Creator/3  "V0"
  Demux/2 -> Bus Creator/2  "Vq"
  Bus Creator/1 -> Vdq0/1
  Vabc/1 -> Park Transform/1
  θm/1 -> Gain3/1
  Park Transform/1 -> Demux/1  "v_dq0"

== system Simulaciones_de_Control/Subsystem Reference1/Sistema Global No Lineal/Transformada Inversa de Park ==
  Idq0 : Inport  OutDataTypeStr=Bus: Idq0
  θm : Inport  Port=2
  Bus Creator : BusCreator  Inputs=3
  Bus Selector : BusSelector  OutputSignals=Id,Iq,I0
  Demux : Demux  Outputs=3
  Gain1 : Gain  Gain=Pp
  Inverse Park Transform : eeTransforms/Inverse Park Transform  AxisAlignment=Q-axis  PowerInvariant=off
      settings: LibrarySourceBlock=|
      | ee_sl_lib/Mathematical
      | Transforms/Inverse
      | Park Transform
  Mux : Mux  Inputs=3
  Iabc : Outport  OutDataTypeStr=Bus: Iabc
  wires:
  Gain1/1 -> Inverse Park Transform/2
  Idq0/1 -> Bus Selector/1
  θm/1 -> Gain1/1
  Demux/1 -> Bus Creator/1  "Ia"
  Inverse Park Transform/1 -> Demux/1  "Iabc"
  Demux/2 -> Bus Creator/2  "Ib"
  Bus Creator/1 -> Iabc/1
  Demux/3 -> Bus Creator/3  "Ic"
  Bus Selector/1 -> Mux/1  "<Id>"
  Bus Selector/2 -> Mux/2  "<Iq>"
  Bus Selector/3 -> Mux/3  "<I0>"
  Mux/1 -> Inverse Park Transform/1

== system Simulaciones_de_Control/Subsystem Reference2/Modulador de Torque Equivalente/Subsystem ==
  T°s : Inport
  Constant1 : Constant  Value=T_sREF
  Constant2 : Constant
  Gain5 : Gain  Gain=alpha_Cu
  Gain6 : Gain  Gain=R_sREF
  Sum3 : Sum  Inputs=+-|
  Sum4 : Sum  Inputs=|++
  R_s : Outport
  wires:
  Sum3/1 -> Gain5/1
  Sum4/1 -> Gain6/1
  Constant2/1 -> Sum4/2
  Constant1/1 -> Sum3/2
  Gain6/1 -> R_s/1  "R_s"
  Gain5/1 -> Sum4/1
  T°s/1 -> Sum3/1

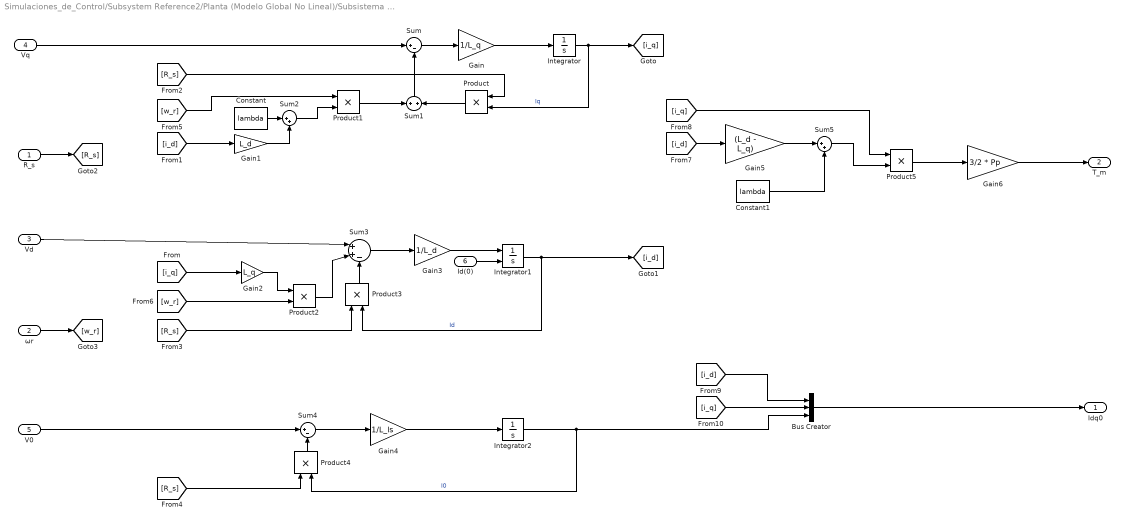
== system Simulaciones_de_Control/Subsystem Reference2/Planta (Modelo Global No Lineal)/Subsistema Electromagnetico ==
  R_s : Inport
  ωr : Inport  Port=2
  Vd : Inport  Port=3
  Vq : Inport  Port=4
  V0 : Inport  Port=5
  Id(0) : Inport  Port=6
  Bus Creator : BusCreator  Inputs=3
  Constant : Constant  Value=lambda
  Constant1 : Constant  Value=lambda
  Gain : Gain  Gain=1/L_q
  Gain1 : Gain  Gain=L_d
  Gain2 : Gain  Gain=L_q
  Gain3 : Gain  Gain=1/L_d
  Gain4 : Gain  Gain=1/L_ls
  Gain5 : Gain  Gain=(L_d - L_q)
  Gain6 : Gain  Gain=3/2 * Pp
  Integrator : Integrator  InitialCondition=init_Iq
  Integrator1 : Integrator  InitialConditionSource=external  InitialCondition=init_Id
  Integrator2 : Integrator  InitialCondition=init_I0
  Product{,1..5} (6 alike) : Product
  Sum : Sum  Inputs=|+-
  Sum1 : Sum
  Sum2 : Sum  Inputs=|++
  Sum3 : Sum  Inputs=|++-
  Sum4 : Sum  Inputs=|+-
  Sum5 : Sum  Inputs=|++
  Idq0 : Outport
  T_m : Outport  Port=2
  wires:
  [i_q] -> Bus Creator/2
  [i_d] -> Bus Creator/1
  Id(0)/1 -> Integrator1/2
  Bus Creator/1 -> Idq0/1
  [i_q] -> Product5/1
  [i_d] -> Gain5/1
  [w_r] -> Product1/1
  ωr/1 -> [w_r]
  [R_s] -> Product4/1
  [R_s] -> Product3/1
  R_s/1 -> [R_s]
  [i_d] -> Gain1/1
  Gain6/1 -> T_m/1
  Product5/1 -> Gain6/1
  Constant1/1 -> Sum5/2
  Integrator1/1 -> Product3/2, [i_d]  "Id"
  Sum5/1 -> Product5/2
  Gain5/1 -> Sum5/1
  V0/1 -> Sum4/1
  Sum4/1 -> Gain4/1
  Gain4/1 -> Integrator2/1
  Integrator2/1 -> Product4/2, Bus Creator/3  "I0"
  Product4/1 -> Sum4/2
  Vd/1 -> Sum3/1
  Sum3/1 -> Gain3/1
  Gain3/1 -> Integrator1/1
  Product3/1 -> Sum3/3
  Gain/1 -> Integrator/1
  Vq/1 -> Sum/1
  Sum/1 -> Gain/1
  Constant/1 -> Sum2/1
  Sum2/1 -> Product1/2
  Gain1/1 -> Sum2/2
  Product1/1 -> Sum1/1
  Sum1/1 -> Sum/2
  Product/1 -> Sum1/2
  [R_s] -> Product/1
  Integrator/1 -> [i_q], Product/2  "Iq"
  [i_q] -> Gain2/1
  Product2/1 -> Sum3/2
  Gain2/1 -> Product2/1
  [w_r] -> Product2/2

== system Simulaciones_de_Control/Subsystem Reference2/Planta (Modelo Global No Lineal)/Subsistema Mecanico Equivalente ==
  note: $\theta_m$
  note: $\omega_m$
  note: $\dot{\omega}_m$
  note: $T_{ld}$
  note: $T_m$
  T_m : Inport
  T_ld : Inport  Port=2
  g : Inport  Port=3
  Gain : Gain  Gain=1/r
  Gain1 : Gain  Gain=b_eq
  Gain2 : Gain  Gain=k_l/r
  Gain3 : Gain  Gain=1/J_eq
  Gain4 : Gain  Gain=1/r
  Integrator : Integrator  InitialCondition=init_w
  Integrator1 : Integrator  InitialCondition=init_theta
  Product : Product
  Sin : Trigonometry
  Sum : Sum  Inputs=|+-
  Sum1 : Sum  Inputs=+++
  ωm : Outport
  θm : Outport  Port=2
  wires:
  Integrator1/1 -> θm/1, Gain4/1
  Integrator/1 -> Gain1/1, Integrator1/1, ωm/1
  g/1 -> Product/1
  Product/1 -> Sum1/2
  T_ld/1 -> Gain/1
  Gain4/1 -> Sin/1
  Gain3/1 -> Integrator/1
  Gain1/1 -> Sum1/3
  Sin/1 -> Gain2/1
  Gain/1 -> Sum1/1
  Gain2/1 -> Product/2
  Sum1/1 -> Sum/2
  T_m/1 -> Sum/1
  Sum/1 -> Gain3/1

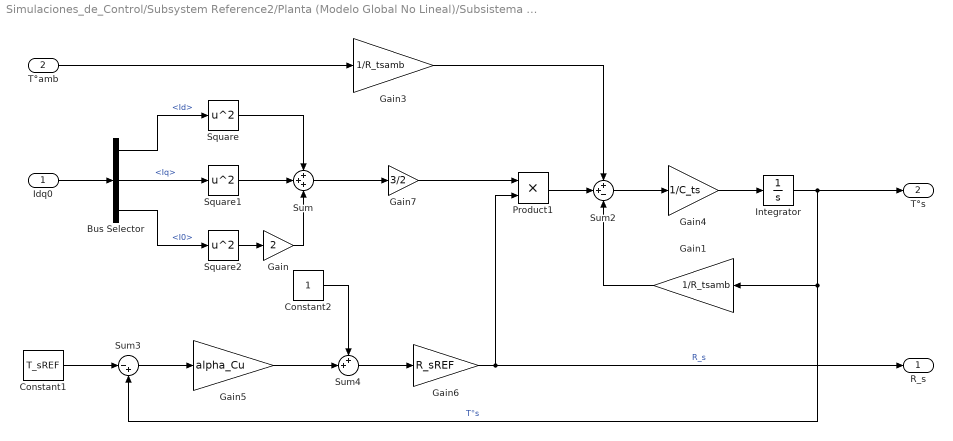
== system Simulaciones_de_Control/Subsystem Reference2/Planta (Modelo Global No Lineal)/Subsistema Termico ==
  Idq0 : Inport
  T°amb : Inport  Port=2
  Bus Selector : BusSelector  OutputSignals=Id,Iq,I0
  Constant1 : Constant  Value=T_sREF
  Constant2 : Constant
  Gain : Gain  Gain=2
  Gain1 : Gain  Gain=1/R_tsamb
  Gain3 : Gain  Gain=1/R_tsamb
  Gain4 : Gain  Gain=1/C_ts
  Gain5 : Gain  Gain=alpha_Cu
  Gain6 : Gain  Gain=R_sREF
  Gain7 : Gain  Gain=3/2
  Integrator : Integrator  InitialCondition=init_Ts
  Product1 : Product
  Square : Math  Operator=square
  Square1 : Math  Operator=square
  Square2 : Math  Operator=square
  Sum : Sum  Inputs=+++
  Sum2 : Sum  Inputs=++-
  Sum3 : Sum  Inputs=|-+
  Sum4 : Sum  Inputs=++|
  R_s : Outport
  T°s : Outport  Port=2
  wires:
  Bus Selector/3 -> Square2/1  "<I0>"
  Bus Selector/1 -> Square/1  "<Id>"
  Constant2/1 -> Sum4/1
  Idq0/1 -> Bus Selector/1
  Gain3/1 -> Sum2/1
  Gain1/1 -> Sum2/3
  Gain4/1 -> Integrator/1
  Product1/1 -> Sum2/2
  Square/1 -> Sum/1
  Sum2/1 -> Gain4/1
  Square2/1 -> Gain/1
  Sum/1 -> Gain7/1
  T°amb/1 -> Gain3/1
  Sum3/1 -> Gain5/1
  Gain5/1 -> Sum4/2
  Gain/1 -> Sum/3
  Constant1/1 -> Sum3/1
  Sum4/1 -> Gain6/1
  Gain7/1 -> Product1/1
  Gain6/1 -> Product1/2, R_s/1  "R_s"
  Integrator/1 -> T°s/1, Gain1/1, Sum3/2  "T°s"
  Square1/1 -> Sum/2
  Bus Selector/2 -> Square1/1  "<Iq>"

== system Simulaciones_de_Control/Subsystem Reference2/Planta (Modelo Global No Lineal)/Transformada Directa de Park ==
  Vabc : Inport  OutDataTypeStr=Bus: Vabc
  θm : Inport  Port=2
  Bus Creator : BusCreator  Inputs=3
  Demux : Demux  Outputs=3
  Gain3 : Gain  Gain=Pp
  MATLAB Function2 : MATLAB Function  Commented=on  TreatAsAtomicUnit=on
  Park Transform : eeTransforms/Park Transform  AxisAlignment=Q-axis  PowerInvariant=off
      settings: LibrarySourceBlock=|
      | ee_sl_lib/Mathematical
      | Transforms/Park Transform
  Vdq0 : Outport  OutDataTypeStr=Bus: Vdq0
  wires:
  Gain3/1 -> Park Transform/2
  Demux/1 -> Bus Creator/1  "Vd"
  Demux/3 -> Bus Creator/3  "V0"
  Demux/2 -> Bus Creator/2  "Vq"
  Bus Creator/1 -> Vdq0/1
  θm/1 -> Gain3/1
  Park Transform/1 -> Demux/1  "v_dq0"
  Vabc/1 -> Park Transform/1

== matlab function Simulaciones_de_Control/Subsystem Reference/Planta (Modelo Global No Lineal)/Transformada Directa de Park/MATLAB Function2 ==
  data: Vabc input; Vdq0 output; theta input
function Vdq0 = TDP_Tension(Vabc, theta)

P = [cos(theta),    cos(theta-2*pi/3),  cos(theta-2*pi/3);...
    sin(theta),     sin(theta-2*pi/3),  sin(theta-2*pi/3);...
    1/2,            1/2,                1/2;];

Vdq0 = 2/3 * P * Vabc;

== matlab function Simulaciones_de_Control/Subsystem Reference2/Planta (Modelo Global No Lineal)/Transformada Directa de Park/MATLAB Function2 ==
  data: Vabc input; Vdq0 output; theta input
function Vdq0 = TDP_Tension(Vabc, theta)

P = [cos(theta),    cos(theta-2*pi/3),  cos(theta-2*pi/3);...
    sin(theta),     sin(theta-2*pi/3),  sin(theta-2*pi/3);...
    1/2,            1/2,                1/2;];

Vdq0 = 2/3 * P * Vabc;

== matlab function Simulaciones_de_Control/Subsystem Reference1/Sistema Global No Lineal/Transformada Directa de Park/MATLAB Function2 ==
  data: Vabc input; Vdq0 output; theta input
function Vdq0 = TDP_Tension(Vabc, theta)

P = [cos(theta),    cos(theta-2*pi/3),  cos(theta-2*pi/3);...
    sin(theta),     sin(theta-2*pi/3),  sin(theta-2*pi/3);...
    1/2,            1/2,                1/2;];

Vdq0 = 2/3 * P * Vabc;
